simulink model "BLDC_SC_fr"  (R2021a)
settings: Solver=VariableStepAuto  StartTime=0.0  StopTime=3.5  MaxStep=1e-5  RelTol=1e-3
undefined symbols (not defined in the file or in its folder): B, DiscIntNeverNeededParam, J, Ke, Ls, p, pm, Rs, sigbuilder_block
libraries: spsVoltageMeasurementLib x3, simulink x1, spsDCVoltageSourceLib x1, spsUniversalBridgeLib x1, spsPermanentMagnetSynchronousMachineLib x1, spspowerguiLib x1
settings Model: SimulationMode=accelerator  Creator=musta  LastModifiedBy=AHMED
settings DebuggingCC: UnderSpecifiedDimensionMsg=warning

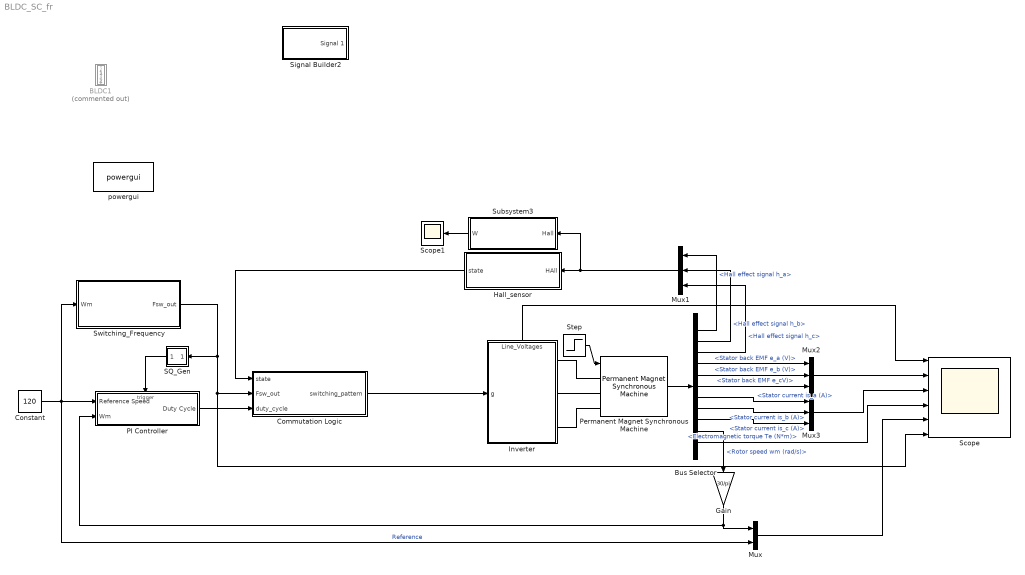
== system BLDC_SC_fr ==
  BLDC1 : Subsystem  Commented=on
  Bus Selector : BusSelector  OutputSignals=Hall effect signal h_a,Hall effect signal h_b,Hall effect signal h_c,Stator back EMF e_a (V),Stator back EMF e_b (V),Stator back EMF e_cV),Stator current is_a (A),Stator current is_b (A),Stator current is_c (A),Rotor speed wm (rad/s),Electromagnetic torque Te (N*m)
  Commutation Logic : Subsystem
  Constant : Constant  Value=120
  Gain : Gain  Gain=30/pi
  Hall_sensor : Subsystem
  Inverter : Subsystem
      settings: PortSchema="{\"entries\":[{\"content\":{\"sides\":[{\"content\":{\"connectorIds\":[\"In1\"]},\"type\":\"ConnectorPlacement.EquallySpacedRectSide\",\"uuid\":\"a4a631f5-5ca6-4816-ae34-76d65d1ebca4\"},{\"content\":{\"connectorIds\":[\"RConn1\",\"RConn2\",\"RConn3\"],\"side\":\"RIGHT\"},\"type\":\"ConnectorPlacement.EquallySpacedRectSide\",\"uuid\":\"fc2fa901-aafd-4005-bc6f-aa03a105cdb5\"},{\"content\":{\"connectorIds\":[\"Out1\"],\"side\":\"TOP\"},\"type\":\"ConnectorPlacement.EquallySpacedRectSide\",\"uuid\":\"9f3df2e4-0b81-43f4-a3b4-b6a902391765\"}]},\"type\":\"ConnectorPlacement.EquallySpacedConnector\",\"uuid\":\"eba0ffe2-2f10-412b-af1b-cd169af8270e\"}],\"packageUris\":[\"http://schema.mathworks.com/mf0/Connector/R2020b\"],\"version\":\"1.0\"}"
  Mux : Mux  Inputs=2
  Mux1 : Mux  Inputs=3
  Mux2 : Mux  Inputs=3
  Mux3 : Mux  Inputs=3
  PI Controller : Subsystem
  Permanent Magnet Synchronous Machine : spsPermanentMagnetSynchronousMachineLib/Permanent Magnet Synchronous Machine  NbPhases=3  FluxDistribution=Trapezoidal  RotorType=Round  MechanicalLoad=Torque Tm  PresetModel=No  ShowDetailedParameters=on  MeasurementBus=off  Resistance=0.1  Inductance=0.0018  dqInductances=[8.5e-3,8.5e-3]  La=0.0018  MachineConstant=Torque Constant (N.m / A_peak)  Flux=0.0034375  VoltageCst=17.2788  TorqueCst=0.165  Flat=120  Mechanical=[0.000621417 0.000303448 24]  PolePairs=4  InitialConditions=[0,0, 0,0]  InitialConditions5ph=[0 0 0 0 0 0]  RefAngle=Aligned with phase A axis (original Park)  IterativeDiscreteModel=Trapezoidal non iterative  TsBlock=-1  TsPowergui=0
  SQ_Gen : Subsystem
  Scope : Scope  NumInputPorts=6
  Scope1 : Scope
  Signal Builder2 : Subsystem  Tag=STV Subsys  LoadFcn=sigbuilder_block('load');  StartFcn=sigbuilder_block('start');  StopFcn=sigbuilder_block('stop');  ClipboardFcn=sigbuilder_block('clipboard');  mask(Sigbuilder block){tuvar=[0:10]}
      mask help: Simulink:masks:SigbuilderBlock_MD
      mask init:
      | if ~strcmp(get_param(bdroot(gcbh),'SimulationStatus'),'stopped') tuvar = sigbuilder_block('maskInit'); end
      settings: CopyFcn=sigbuilder_block('copy');  DeleteFcn=sigbuilder_block('delete');  ModelCloseFcn=sigbuilder_block('modelClose');  PreSaveFcn=sigbuilder_block('preSave');  PauseFcn=sigbuilder_block('pause');  ContinueFcn=sigbuilder_block('continue');  NameChangeFcn=sigbuilder_block('namechange');  OpenFcn=sigbuilder_block('open',[5.4 30 1141.2 522.6 ]);  CloseFcn=sigbuilder_block('close');
      mask Display: plot(0, 0, 100, 100,[2, 2, 32, 32, 2], [68, 8, 8, 68, 68],[32, 2], [38, 38], [32, 19, 2],[53, 60, 44], [32, 17, 17, 2],[16, 16, 31, 31]);txt = getActiveGroup(gcbh);text(2, 100, txt,'verticalAlignment', 'top');
  Step : Step  Time=1.25  After=0  SampleTime=0
  Subsystem3 : Subsystem
  Switching_Frequency : Subsystem
  powergui : spspowerguiLib/powergui  Priority=1  SimulationMode=Continuous  SampleTime=1e-6  frequency=60  Iterations=50  frequencyindice=0  Pbase=100e6  ErrMax=1e-4  UnitsV=kV  UnitsW=MW  buscounter=0  FunctionMessages=off  echomessages=off  EnableUseOfTLC=off  CurrentSourceSwitches=off  DisableSnubberDevices=off  DisableRonSwitches=off  DisableVfSwitches=off  DisplayEquations=off  AutomaticDiscreteSolvers=off  SolverType=Tustin/Backward Euler (TBE)  Interpol=off  ExternalGateDelay=off  methode=off  Ts=100  x0status=blocks  SPID=on  SwTol=0  HookPort=off  NonlinearTolerance=1e-4  nMaxIteration=100  ContinueOnMaxIteration=off  RestoreLinks=warning  ResistiveCurrentMeasurement=off  Frange=[0:2:500]  Ylog=off  Xlog=on  ShowGrid=off  save=off  variable=ZData  structure=0  ZoomFFT=off  StartTime=0.0  cycles=1  DisplayStyle=1  fundamental=60  FreqAxis=off  MaxFrequency=1000  frequencyindicesteady=1  RmsSteady=1  display=off
  wires:
  Hall_sensor/1(state) -> Commutation Logic/1("state ")
  PI Controller/1(Duty Cycle) -> Commutation Logic/3(duty_cycle)
  Switching_Frequency/1(Fsw_out) -> Scope/6, Commutation Logic/2(Fsw_out), SQ_Gen/1(Input)
  SQ_Gen/1(Cs) -> PI Controller/Trigger
  Permanent Magnet Synchronous Machine/1 -> Bus Selector/1
  Bus Selector/1 -> Mux1/1  "<Hall effect signal h_a>"
  Bus Selector/2 -> Mux1/2  "<Hall effect signal h_b>"
  Bus Selector/3 -> Mux1/3  "<Hall effect signal h_c>"
  Bus Selector/4 -> Mux2/1  "<Stator back EMF e_a (V)>"
  Bus Selector/5 -> Mux2/2  "<Stator back EMF e_b (V)>"
  Bus Selector/6 -> Mux2/3  "<Stator back EMF e_cV)>"
  Mux2/1 -> Scope/2
  Bus Selector/7 -> Mux3/1  "<Stator current is_a (A)>"
  Bus Selector/8 -> Mux3/2  "<Stator current is_b (A)>"
  Bus Selector/9 -> Mux3/3  "<Stator current is_c (A)>"
  Mux3/1 -> Scope/3
  Bus Selector/10 -> Gain/1  "<Rotor speed wm (rad/s)>"
  Bus Selector/11 -> Scope/4  "<Electromagnetic torque Te (N*m)>"
  Mux/1 -> Scope/5
  Step/1 -> Permanent Magnet Synchronous Machine/1
  Inverter/1(Line_Voltages) -> Scope/1
  Commutation Logic/1("  switching_pattern") -> Inverter/1(g)
  Constant/1 -> Switching_Frequency/1(Wm), Mux/2, PI Controller/1(Reference Speed)  "Reference"
  Mux1/1 -> Subsystem3/1(Hall), Hall_sensor/1(HAll)
  Gain/1 -> PI Controller/2(Wm), Mux/1
  Subsystem3/1(W) -> Scope1/1
  connections:
  Inverter/RConn1 -- Permanent Magnet Synchronous Machine/LConn1
  Inverter/RConn2 -- Permanent Magnet Synchronous Machine/LConn2
  Inverter/RConn3 -- Permanent Magnet Synchronous Machine/LConn3

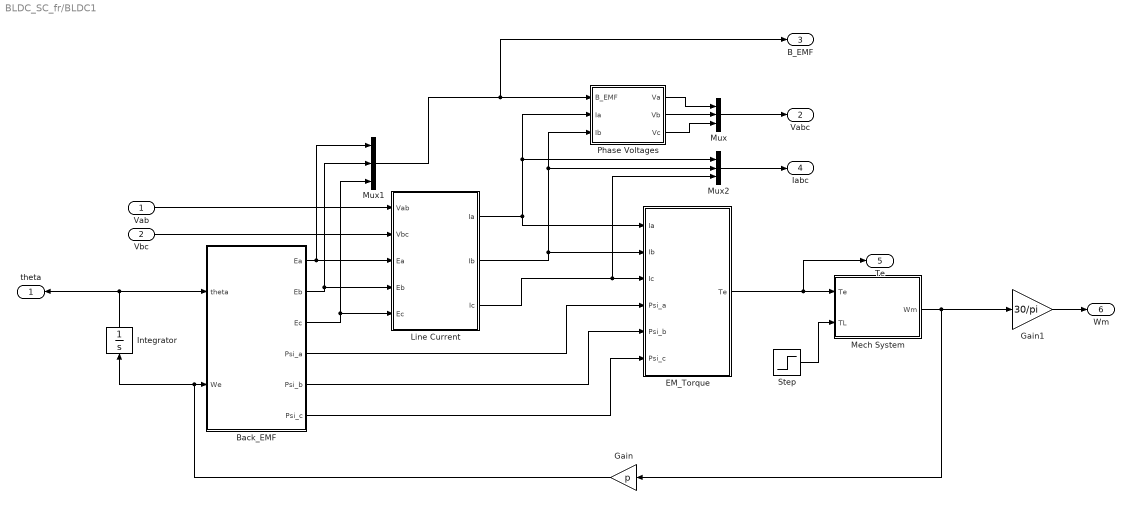
== system BLDC_SC_fr/BLDC1 ==
  Vab : Inport
  Vbc : Inport  Port=2
  Back_EMF : Subsystem
  EM_Torque : Subsystem
  Gain : Gain  Gain=p
  Gain1 : Gain  Gain=30/pi
  Integrator : Integrator
  Line Current : Subsystem
  Mech System : Subsystem
  Mux : Mux  Inputs=3
  Mux1 : Mux  Inputs=3
  Mux2 : Mux  Inputs=3
  Phase Voltages : Subsystem
  Step : Step  Time=2.5  Before=0.5  After=1.5  SampleTime=0
  theta : Outport
  Vabc : Outport  Port=2
  B_EMF : Outport  Port=3
  Iabc : Outport  Port=4
  Te : Outport  Port=5
  Wm : Outport  Port=6
  wires:
  Integrator/1 -> Back_EMF/1(theta), theta/1
  Mux2/1 -> Iabc/1
  Mux/1 -> Vabc/1
  Phase Voltages/3(Vc) -> Mux/3
  Phase Voltages/2(Vb) -> Mux/2
  Phase Voltages/1(Va) -> Mux/1
  Line Current/1(Ia) -> Phase Voltages/2(Ia), Mux2/1, EM_Torque/1(Ia)
  Gain1/1 -> Wm/1
  Vbc/1 -> Line Current/2(Vbc)
  Step/1 -> Mech System/2(TL)
  Vab/1 -> Line Current/1(Vab)
  Mux1/1 -> Phase Voltages/1(B_EMF), B_EMF/1
  Back_EMF/4(Psi_a) -> EM_Torque/4(Psi_a)
  Line Current/2(Ib) -> EM_Torque/2(Ib), Phase Voltages/3(Ib), Mux2/2
  Back_EMF/5(Psi_b) -> EM_Torque/5(Psi_b)
  Gain/1 -> Back_EMF/2(We), Integrator/1
  Back_EMF/6(Psi_c) -> EM_Torque/6(Psi_c)
  EM_Torque/1(Te) -> Mech System/1(Te), Te/1
  Back_EMF/2(Eb) -> Line Current/4(Eb), Mux1/2
  Back_EMF/3(Ec) -> Mux1/3, Line Current/5(Ec)
  Line Current/3(Ic) -> EM_Torque/3(Ic), Mux2/3
  Back_EMF/1(Ea) -> Line Current/3(Ea), Mux1/1
  Mech System/1(Wm) -> Gain/1, Gain1/1

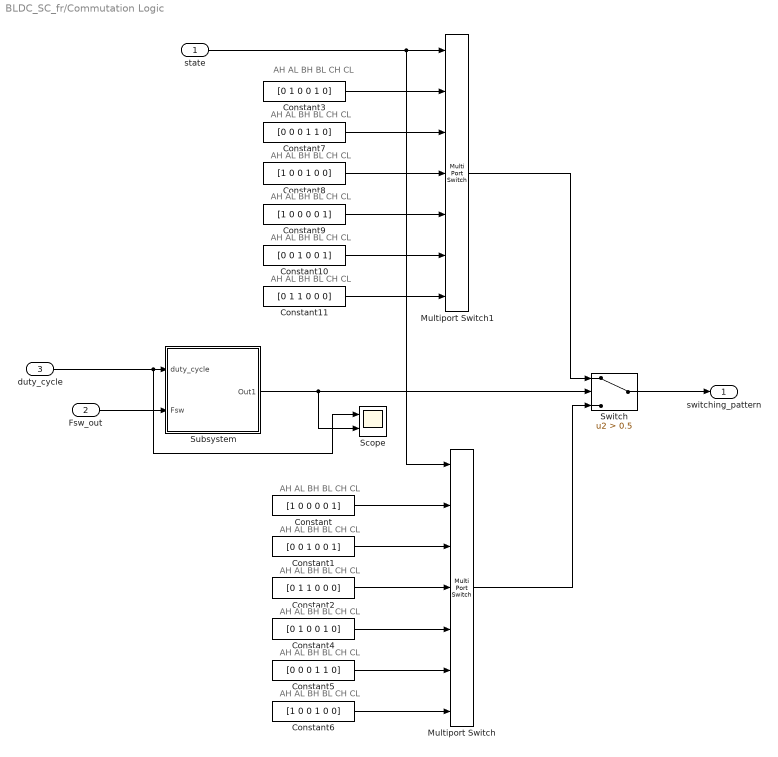
== system BLDC_SC_fr/Commutation Logic ==
  note: AH AL BH BL CH CL
  note: AH AL BH BL CH CL
  note: AH AL BH BL CH CL
  note: AH AL BH BL CH CL
  note: AH AL BH BL CH CL
  note: AH AL BH BL CH CL
  note: AH AL BH BL CH CL
  note: AH AL BH BL CH CL
  note: AH AL BH BL CH CL
  note: AH AL BH BL CH CL
  note: AH AL BH BL CH CL
  note: AH AL BH BL CH CL
  "state " : Inport
  Fsw_out : Inport  Port=2
  duty_cycle : Inport  Port=3
  Constant : Constant  Value=[1 0 0 0 0 1]
  Constant1 : Constant  Value=[0 0 1 0 0 1]
  Constant10 : Constant  Value=[0 0 1 0 0 1]
  Constant11 : Constant  Value=[0 1 1 0 0 0]
  Constant2 : Constant  Value=[0 1 1 0 0 0]
  Constant3 : Constant  Value=[0 1 0 0 1 0]
  Constant4 : Constant  Value=[0 1 0 0 1 0]
  Constant5 : Constant  Value=[0 0 0 1 1 0]
  Constant6 : Constant  Value=[1 0 0 1 0 0]
  Constant7 : Constant  Value=[0 0 0 1 1 0]
  Constant8 : Constant  Value=[1 0 0 1 0 0]
  Constant9 : Constant  Value=[1 0 0 0 0 1]
  Multiport Switch : MultiPortSwitch  Inputs=6
  Multiport Switch1 : MultiPortSwitch  Inputs=6
  Scope : Scope  NumInputPorts=2
  Subsystem : Subsystem
  Switch : Switch  Criteria=u2 > Threshold  Threshold=0.5
  "  switching_pattern" : Outport  VectorParamsAs1DForOutWhenUnconnected=off
  wires:
  Constant1/1 -> Multiport Switch/3
  Constant11/1 -> Multiport Switch1/7
  Constant2/1 -> Multiport Switch/4
  Constant10/1 -> Multiport Switch1/6
  Constant/1 -> Multiport Switch/2
  Switch/1 -> "  switching_pattern"/1
  Constant9/1 -> Multiport Switch1/5
  Constant7/1 -> Multiport Switch1/3
  Constant6/1 -> Multiport Switch/7
  Constant3/1 -> Multiport Switch1/2
  Constant8/1 -> Multiport Switch1/4
  Constant4/1 -> Multiport Switch/5
  Constant5/1 -> Multiport Switch/6
  "state "/1 -> Multiport Switch/1, Multiport Switch1/1
  Multiport Switch1/1 -> Switch/1
  Multiport Switch/1 -> Switch/3
  duty_cycle/1 -> Scope/1, Subsystem/1(duty_cycle)
  Fsw_out/1 -> Subsystem/2(Fsw)
  Subsystem/1(Out1) -> Scope/2, Switch/2

== system BLDC_SC_fr/Hall_sensor ==
  HAll : Inport
  Demux : Demux  Outputs=3
  MATLAB Function : MATLAB Function  TreatAsAtomicUnit=on
  state : Outport
  wires:
  HAll/1 -> Demux/1
  Demux/1 -> MATLAB Function/1(H1)
  Demux/2 -> MATLAB Function/2(H2)
  Demux/3 -> MATLAB Function/3(H3)
  MATLAB Function/1(State) -> state/1

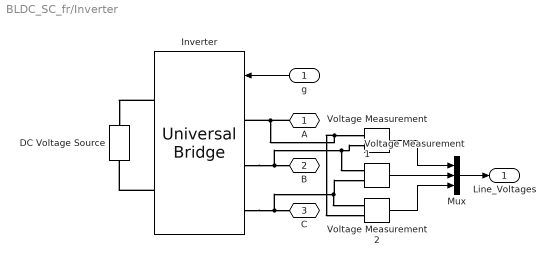
== system BLDC_SC_fr/Inverter ==
  g : Inport
  DC Voltage Source : spsDCVoltageSourceLib/DC Voltage Source  Amplitude=48  Measurements=None
  Inverter : spsUniversalBridgeLib/Universal Bridge  Arms=3  SnubberResistance=1e5  SnubberCapacitance=inf  Device=IGBT / Diodes  Ron=1e-3  Lon=0  ForwardVoltages="[  0  0  ]"  ForwardVoltage=0  GTOparameters=[ 10e-6 , 20e-6 ]  IGBTparameters=[ 1e-6 , 2e-6 ]  Measurements=None  Measurements_2=None  converterType=Rectifier
  Mux : Mux  Inputs=3
  Voltage Measurement : spsVoltageMeasurementLib/Voltage Measurement  PhasorSimulation=off  OutputType=Complex  PSBequivalent=0
  Voltage Measurement1 : spsVoltageMeasurementLib/Voltage Measurement  PhasorSimulation=off  OutputType=Complex  PSBequivalent=0
  Voltage Measurement2 : spsVoltageMeasurementLib/Voltage Measurement  PhasorSimulation=off  OutputType=Complex  PSBequivalent=0
  A : PMIOPort  Side=Right
  B : PMIOPort  Port=2  Side=Right
  C : PMIOPort  Port=3  Side=Right
  Line_Voltages : Outport
  wires:
  g/1 -> Inverter/1
  Voltage Measurement/1 -> Mux/1
  Voltage Measurement1/1 -> Mux/2
  Voltage Measurement2/1 -> Mux/3
  Mux/1 -> Line_Voltages/1
  connections:
  Inverter/RConn1 -- DC Voltage Source/RConn1
  Inverter/RConn2 -- DC Voltage Source/LConn1
  A/RConn1 -- Voltage Measurement/LConn1 -- Voltage Measurement2/LConn2 -- Inverter/LConn1
  Inverter/LConn2 -- Voltage Measurement1/LConn1 -- Voltage Measurement/LConn2 -- B/RConn1
  Inverter/LConn3 -- Voltage Measurement2/LConn1 -- Voltage Measurement1/LConn2 -- C/RConn1

== system BLDC_SC_fr/PI Controller ==
  Reference Speed : Inport
  Wm : Inport  Port=2
  Trigger : TriggerPort  VariantControl=(inherit)  PortDimensions=1
  PI_system3 : Subsystem
  Sum : Sum  Inputs=|+-
  Duty Cycle : Outport
  wires:
  Sum/1 -> PI_system3/1(Error)
  PI_system3/1(T_ref) -> Duty Cycle/1
  Wm/1 -> Sum/2
  Reference Speed/1 -> Sum/1

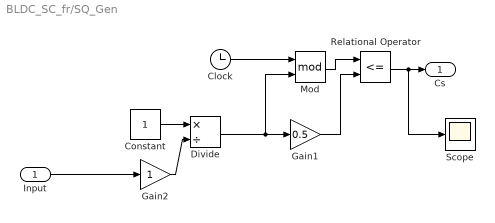
== system BLDC_SC_fr/SQ_Gen ==
  Input : Inport
  Clock : Clock
  Constant : Constant
  Divide : Product  Inputs=*/
  Gain1 : Gain  Gain=0.5
  Gain2 : Gain
  Mod : Math  Operator=mod  SaturateOnIntegerOverflow=on
  Relational Operator : RelationalOperator  Operator=<=  OutDataTypeStr=boolean  RndMeth=Simplest
  Scope : Scope
  Cs : Outport
  wires:
  Input/1 -> Gain2/1
  Clock/1 -> Mod/1
  Mod/1 -> Relational Operator/1
  Gain2/1 -> Divide/2
  Divide/1 -> Gain1/1, Mod/2
  Constant/1 -> Divide/1
  Gain1/1 -> Relational Operator/2
  Relational Operator/1 -> Scope/1, Cs/1

== system BLDC_SC_fr/Signal Builder2 ==
  Demux : Demux  Tag=STV Demux  Outputs=1
      settings: DisplayOption=none
  FromWs : FromWorkspace  Tag=STV FromWs  VariableName=tuvar  SampleTime=-1
      SigBuilderData=|
      | common.afterFinalStr = 'Extrapolate'
      | common.sampleTime = '-1'
      | dataSet.timeRange = [0 3.5]
      | dataSet.name = 'Group 1'
      | sbobj.Groups.Name = 'Group 1'
      | sbobj.Groups.Signals.Name = 'Signal 1'
      | sbobj.Groups.Signals.XData = [0 0.25 0.5 1 1.5 1.75 2 2.5 2.75 3 3.5]
      | sbobj.Groups.Signals.YData = [0.25 0.5 0.5 1.5 1.5 2 1.5 1.5 0.5 0.25 0.25]
      | sbobj.Groups.TimeRange = [0 3.5]
  Signal 1 : Outport  Tag=STV Outport
  wires:
  FromWs/1 -> Demux/1
  Demux/1 -> Signal 1/1

== system BLDC_SC_fr/Subsystem3 ==
  Hall : Inport
  Add : Sum  Inputs=+++
  Demux : Demux  Outputs=3
  Gain2 : Gain  Gain=1/3
  Scope1 : Scope  NumInputPorts=4
  Subsystem : Subsystem
  Subsystem1 : Subsystem
  Subsystem2 : Subsystem
  W : Outport
  wires:
  Subsystem2/1(Out1) -> Add/1
  Demux/3 -> Subsystem/1(U)
  Subsystem/1(Out1) -> Add/3
  Demux/2 -> Subsystem1/1(U)
  Add/1 -> Gain2/1
  Subsystem1/1(Out1) -> Add/2
  Demux/1 -> Subsystem2/1(U)
  Hall/1 -> Demux/1
  Gain2/1 -> W/1

== system BLDC_SC_fr/Switching_Frequency ==
  Wm : Inport
  Gain : Gain  Gain=10
  Gain1 : Gain  Gain=1/500
  Gain2 : Gain  Gain=500
  N2F : Gain  Gain=48/120
  Round : Rounding  Operator=round
  Saturation : Saturate  UpperLimit=10000  LowerLimit=4000
  Wm2N : Gain  Gain=60/(2*pi)
  Fsw_out : Outport
  wires:
  Wm2N/1 -> N2F/1
  Wm/1 -> Wm2N/1
  N2F/1 -> Gain/1
  Saturation/1 -> Gain1/1
  Gain1/1 -> Round/1
  Gain2/1 -> Fsw_out/1
  Round/1 -> Gain2/1
  Gain/1 -> Saturation/1

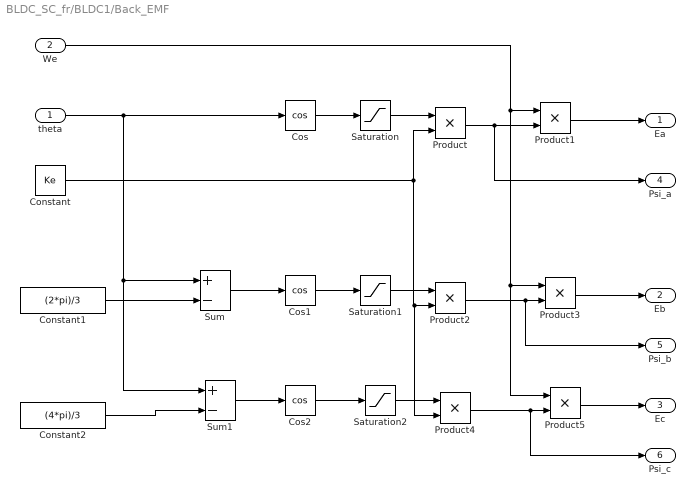
== system BLDC_SC_fr/BLDC1/Back_EMF ==
  theta : Inport
  We : Inport  Port=2
  Constant : Constant  Value=Ke
  Constant1 : Constant  Value=(2*pi)/3
  Constant2 : Constant  Value=(4*pi)/3
  Cos : Trigonometry  Operator=cos
  Cos1 : Trigonometry  Operator=cos
  Cos2 : Trigonometry  Operator=cos
  Product{,1..5} (6 alike) : Product
  Saturation : Saturate
  Saturation1 : Saturate
  Saturation2 : Saturate
  Sum : Sum  Inputs=+-
  Sum1 : Sum  Inputs=+-
  Ea : Outport
  Eb : Outport  Port=2
  Ec : Outport  Port=3
  Psi_a : Outport  Port=4
  Psi_b : Outport  Port=5
  Psi_c : Outport  Port=6
  wires:
  Product5/1 -> Ec/1
  Constant2/1 -> Sum1/2
  Sum1/1 -> Cos2/1
  Cos2/1 -> Saturation2/1
  Saturation2/1 -> Product4/1
  Product4/1 -> Product5/2, Psi_c/1
  Product3/1 -> Eb/1
  Product2/1 -> Product3/2, Psi_b/1
  Saturation1/1 -> Product2/1
  Cos1/1 -> Saturation1/1
  Sum/1 -> Cos1/1
  Constant1/1 -> Sum/2
  Constant/1 -> Product/2, Product2/2, Product4/2
  Product1/1 -> Ea/1
  We/1 -> Product1/1, Product3/1, Product5/1
  Product/1 -> Product1/2, Psi_a/1
  Saturation/1 -> Product/1
  Cos/1 -> Saturation/1
  theta/1 -> Sum/1, Sum1/1, Cos/1

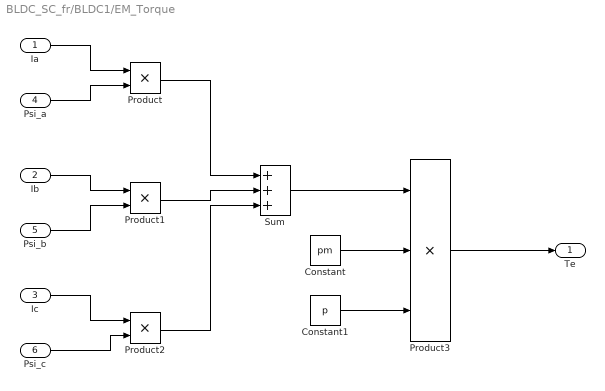
== system BLDC_SC_fr/BLDC1/EM_Torque ==
  Ia : Inport
  Ib : Inport  Port=2
  Ic : Inport  Port=3
  Psi_a : Inport  Port=4
  Psi_b : Inport  Port=5
  Psi_c : Inport  Port=6
  Constant : Constant  Value=pm
  Constant1 : Constant  Value=p
  Product : Product
  Product1 : Product
  Product2 : Product
  Product3 : Product  Inputs=3
  Sum : Sum  Inputs=+++
  Te : Outport
  wires:
  Product3/1 -> Te/1
  Constant1/1 -> Product3/3
  Constant/1 -> Product3/2
  Sum/1 -> Product3/1
  Product2/1 -> Sum/3
  Product1/1 -> Sum/2
  Product/1 -> Sum/1
  Psi_c/1 -> Product2/2
  Ic/1 -> Product2/1
  Psi_b/1 -> Product1/2
  Ib/1 -> Product1/1
  Psi_a/1 -> Product/2
  Ia/1 -> Product/1

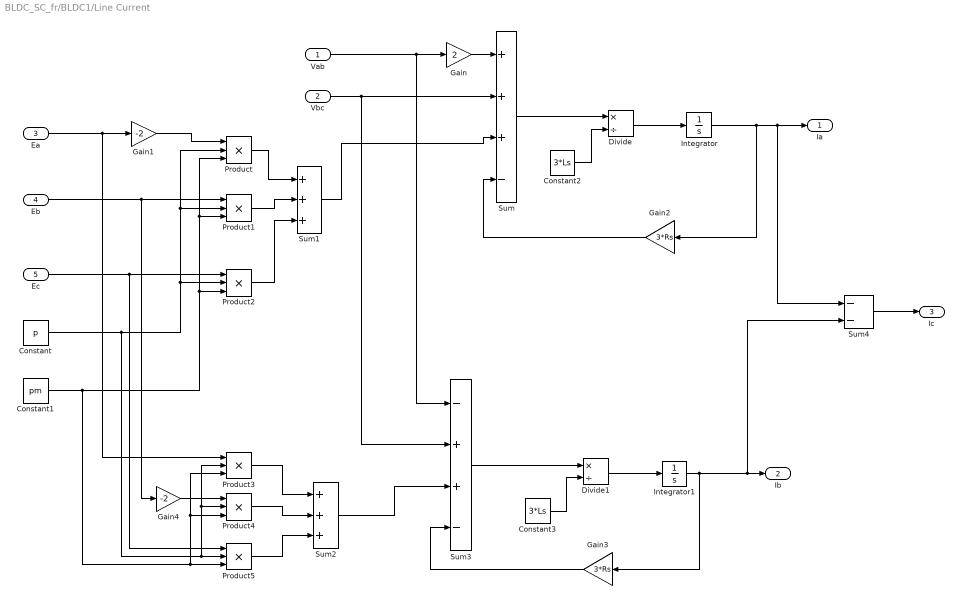
== system BLDC_SC_fr/BLDC1/Line Current ==
  Vab : Inport
  Vbc : Inport  Port=2
  Ea : Inport  Port=3
  Eb : Inport  Port=4
  Ec : Inport  Port=5
  Constant : Constant  Value=p
  Constant1 : Constant  Value=pm
  Constant2 : Constant  Value=3*Ls
  Constant3 : Constant  Value=3*Ls
  Divide : Product  Inputs=*/
  Divide1 : Product  Inputs=*/
  Gain : Gain  Gain=2
  Gain1 : Gain  Gain=-2
  Gain2 : Gain  Gain=3*Rs
  Gain3 : Gain  Gain=3*Rs
  Gain4 : Gain  Gain=-2
  Integrator : Integrator
  Integrator1 : Integrator
  Product{,1..5} (6 alike) : Product  Inputs=3
  Sum : Sum  Inputs=+++-
  Sum1 : Sum  Inputs=+++
  Sum2 : Sum  Inputs=+++
  Sum3 : Sum  Inputs=-++-
  Sum4 : Sum  Inputs=--
  Ia : Outport
  Ib : Outport  Port=2
  Ic : Outport  Port=3
  wires:
  Gain4/1 -> Product4/1
  Sum4/1 -> Ic/1
  Gain3/1 -> Sum3/4
  Integrator1/1 -> Ib/1, Sum4/2, Gain3/1
  Sum3/1 -> Divide1/1
  Constant3/1 -> Divide1/2
  Divide1/1 -> Integrator1/1
  Sum2/1 -> Sum3/3
  Product5/1 -> Sum2/3
  Product4/1 -> Sum2/2
  Product3/1 -> Sum2/1
  Gain2/1 -> Sum/4
  Integrator/1 -> Ia/1, Sum4/1, Gain2/1
  Divide/1 -> Integrator/1
  Constant2/1 -> Divide/2
  Sum/1 -> Divide/1
  Sum1/1 -> Sum/3
  Product2/1 -> Sum1/3
  Product1/1 -> Sum1/2
  Product/1 -> Sum1/1
  Constant1/1 -> Product2/3, Product/3, Product1/3, Product5/3, Product4/3, Product3/3
  Constant/1 -> Product2/2, Product/2, Product1/2, Product5/2, Product4/2, Product3/2
  Ec/1 -> Product2/1, Product5/1
  Eb/1 -> Product1/1, Gain4/1
  Gain1/1 -> Product/1
  Ea/1 -> Gain1/1, Product3/1
  Vbc/1 -> Sum/2, Sum3/2
  Gain/1 -> Sum/1
  Vab/1 -> Gain/1, Sum3/1

== system BLDC_SC_fr/BLDC1/Mech System ==
  Te : Inport
  TL : Inport  Port=2
  Constant : Constant  Value=J
  Divide : Product  Inputs=*/
  Gain : Gain  Gain=B
  Integrator : Integrator
  Sum : Sum  Inputs=+--
  Wm : Outport
  wires:
  Gain/1 -> Sum/3
  Integrator/1 -> Wm/1, Gain/1
  Divide/1 -> Integrator/1
  Constant/1 -> Divide/2
  Sum/1 -> Divide/1
  TL/1 -> Sum/2
  Te/1 -> Sum/1

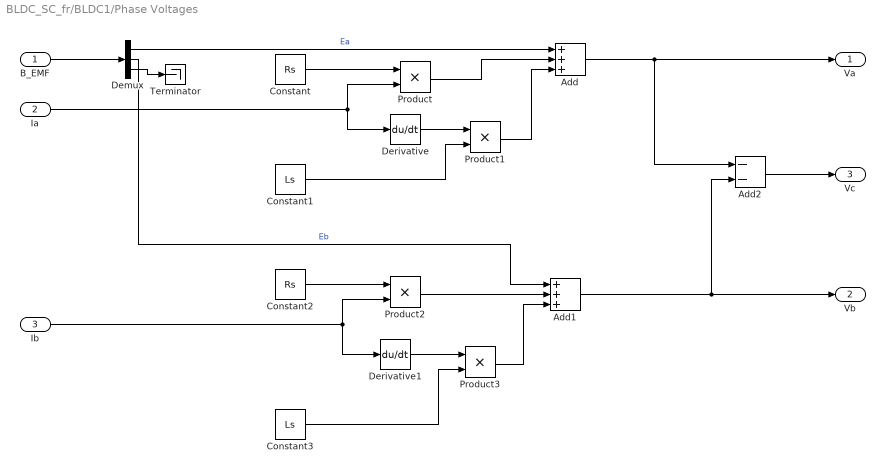
== system BLDC_SC_fr/BLDC1/Phase Voltages ==
  B_EMF : Inport
  Ia : Inport  Port=2
  Ib : Inport  Port=3
  Add : Sum  Inputs=+++
  Add1 : Sum  Inputs=+++
  Add2 : Sum  Inputs=--
  Constant : Constant  Value=Rs
  Constant1 : Constant  Value=Ls
  Constant2 : Constant  Value=Rs
  Constant3 : Constant  Value=Ls
  Demux : Demux  Outputs=3
  Derivative : Derivative
  Derivative1 : Derivative
  Product{,1..3} (4 alike) : Product
  Terminator : Terminator
  Va : Outport
  Vb : Outport  Port=2
  Vc : Outport  Port=3
  wires:
  Add2/1 -> Vc/1
  Constant3/1 -> Product3/2
  Constant2/1 -> Product2/1
  Constant1/1 -> Product1/2
  Constant/1 -> Product/1
  Demux/3 -> Terminator/1
  Add1/1 -> Vb/1, Add2/2
  Demux/2 -> Add1/1  "Eb"
  Product2/1 -> Add1/2
  Derivative1/1 -> Product3/1
  Product3/1 -> Add1/3
  Ib/1 -> Product2/2, Derivative1/1
  Demux/1 -> Add/1  "Ea"
  B_EMF/1 -> Demux/1
  Ia/1 -> Product/2, Derivative/1
  Product1/1 -> Add/3
  Add/1 -> Va/1, Add2/1
  Derivative/1 -> Product1/1
  Product/1 -> Add/2

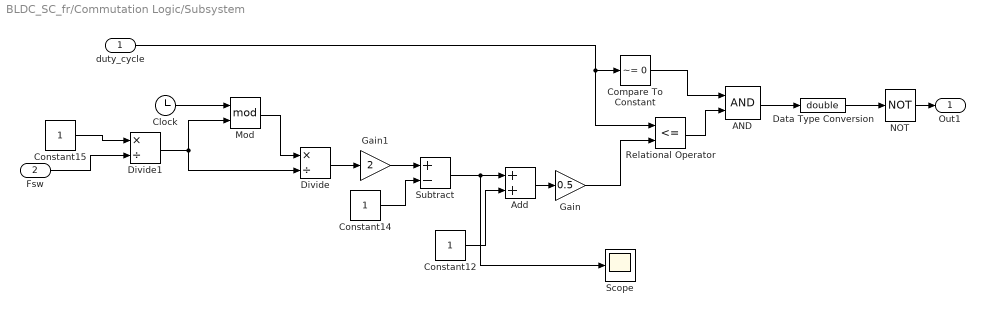
== system BLDC_SC_fr/Commutation Logic/Subsystem ==
  duty_cycle : Inport
  Fsw : Inport  Port=2
  AND : Logic  AllPortsSameDT=off  OutDataTypeStr=boolean
  Add : Sum
  Clock : Clock
  Compare To Constant : simulink/Logic and Bit Operations/Compare To Constant  relop=~=  const=0  OutDataTypeStr=boolean
  Constant12 : Constant
  Constant14 : Constant
  Constant15 : Constant
  Data Type Conversion : DataTypeConversion  OutDataTypeStr=double
  Divide : Product  Inputs=*/
  Divide1 : Product  Inputs=*/
  Gain : Gain  Gain=0.5
  Gain1 : Gain  Gain=2
  Mod : Math  Operator=mod  SaturateOnIntegerOverflow=on
  NOT : Logic  Operator=NOT  IconShape=distinctive  AllPortsSameDT=off  OutDataTypeStr=boolean
  Relational Operator : RelationalOperator  Operator=<=  OutDataTypeStr=boolean  RndMeth=Simplest
  Scope : Scope
  Subtract : Sum  Inputs=+-
  Out1 : Outport
  wires:
  Constant12/1 -> Add/2
  Add/1 -> Gain/1
  Relational Operator/1 -> AND/2
  Constant14/1 -> Subtract/2
  NOT/1 -> Out1/1
  duty_cycle/1 -> Relational Operator/1, Compare To Constant/1
  Subtract/1 -> Scope/1, Add/1
  Compare To Constant/1 -> AND/1
  Gain/1 -> Relational Operator/2
  AND/1 -> Data Type Conversion/1
  Divide1/1 -> Divide/2, Mod/2
  Gain1/1 -> Subtract/1
  Clock/1 -> Mod/1
  Mod/1 -> Divide/1
  Divide/1 -> Gain1/1
  Constant15/1 -> Divide1/1
  Fsw/1 -> Divide1/2
  Data Type Conversion/1 -> NOT/1

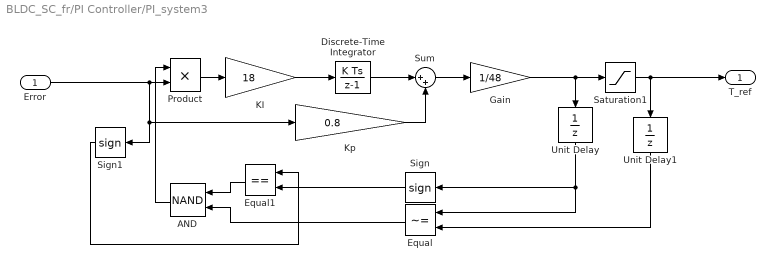
== system BLDC_SC_fr/PI Controller/PI_system3 ==
  Error : Inport
  AND : Logic  Operator=NAND  AllPortsSameDT=off  OutDataTypeStr=boolean
  Discrete-Time Integrator : DiscreteIntegrator  SampleTime=-1  ICPrevOutput=DiscIntNeverNeededParam  ICPrevScaledInput=DiscIntNeverNeededParam
  Equal : RelationalOperator  Operator=~=  OutDataTypeStr=boolean  RndMeth=Simplest
  Equal1 : RelationalOperator  Operator===  OutDataTypeStr=boolean  RndMeth=Simplest
  Gain : Gain  Gain=1/48
  KI : Gain  Gain=18
  Kp : Gain  Gain=0.8
  Product : Product
  Saturation1 : Saturate  UpperLimit=1  LowerLimit=0
  Sign : Signum
  Sign1 : Signum
  Sum : Sum  Inputs=|++
  Unit Delay : UnitDelay  SampleTime=-1  HasFrameUpgradeWarning=on
  Unit Delay1 : UnitDelay  SampleTime=-1  HasFrameUpgradeWarning=on
  T_ref : Outport
  wires:
  Error/1 -> Kp/1, Sign1/1, Product/2
  AND/1 -> Product/1
  Unit Delay1/1 -> Equal/2
  Product/1 -> KI/1
  Unit Delay/1 -> Equal/1, Sign/1
  Equal/1 -> AND/2
  Equal1/1 -> AND/1
  Sign1/1 -> Equal1/1
  Sign/1 -> Equal1/2
  Saturation1/1 -> Unit Delay1/1, T_ref/1
  Sum/1 -> Gain/1
  KI/1 -> Discrete-Time Integrator/1
  Kp/1 -> Sum/2
  Discrete-Time Integrator/1 -> Sum/1
  Gain/1 -> Saturation1/1, Unit Delay/1

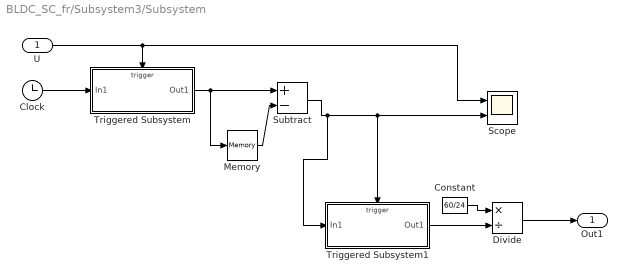
== system BLDC_SC_fr/Subsystem3/Subsystem ==
  U : Inport
  Clock : Clock
  Constant : Constant  Value=60/24
  Divide : Product  Inputs=*/
  Memory : Memory  InheritSampleTime=on
  Scope : Scope  NumInputPorts=2
  Subtract : Sum  Inputs=+-
  Triggered Subsystem : Subsystem  TreatAsAtomicUnit=on
  Triggered Subsystem1 : Subsystem  TreatAsAtomicUnit=on
  Out1 : Outport
  wires:
  Clock/1 -> Triggered Subsystem/1(In1)
  Subtract/1 -> Triggered Subsystem1/1(In1), Triggered Subsystem1/Trigger, Scope/2
  Triggered Subsystem/1(Out1) -> Subtract/1, Memory/1
  Memory/1 -> Subtract/2
  U/1 -> Triggered Subsystem/Trigger, Scope/1
  Triggered Subsystem1/1(Out1) -> Divide/2
  Constant/1 -> Divide/1
  Divide/1 -> Out1/1

== system BLDC_SC_fr/Subsystem3/Subsystem1 ==
  U : Inport
  Clock : Clock
  Constant : Constant  Value=60/24
  Divide : Product  Inputs=*/
  Memory : Memory  InheritSampleTime=on
  Scope : Scope  NumInputPorts=2
  Subtract : Sum  Inputs=+-
  Triggered Subsystem : Subsystem  TreatAsAtomicUnit=on
  Triggered Subsystem1 : Subsystem  TreatAsAtomicUnit=on
  Out1 : Outport
  wires:
  Divide/1 -> Out1/1
  Constant/1 -> Divide/1
  Triggered Subsystem1/1(Out1) -> Divide/2
  U/1 -> Scope/1, Triggered Subsystem/Trigger
  Memory/1 -> Subtract/2
  Triggered Subsystem/1(Out1) -> Memory/1, Subtract/1
  Subtract/1 -> Scope/2, Triggered Subsystem1/Trigger, Triggered Subsystem1/1(In1)
  Clock/1 -> Triggered Subsystem/1(In1)

== system BLDC_SC_fr/Subsystem3/Subsystem2 ==
  U : Inport
  Clock : Clock
  Constant : Constant  Value=60/24
  Divide : Product  Inputs=*/
  Memory : Memory  InheritSampleTime=on
  Scope : Scope  NumInputPorts=2
  Subtract : Sum  Inputs=+-
  Triggered Subsystem : Subsystem  TreatAsAtomicUnit=on
  Triggered Subsystem1 : Subsystem  TreatAsAtomicUnit=on
  Out1 : Outport
  wires:
  Clock/1 -> Triggered Subsystem/1(In1)
  Subtract/1 -> Triggered Subsystem1/1(In1), Triggered Subsystem1/Trigger, Scope/2
  Triggered Subsystem/1(Out1) -> Subtract/1, Memory/1
  Memory/1 -> Subtract/2
  U/1 -> Triggered Subsystem/Trigger, Scope/1
  Triggered Subsystem1/1(Out1) -> Divide/2
  Constant/1 -> Divide/1
  Divide/1 -> Out1/1

== system BLDC_SC_fr/Subsystem3/Subsystem/Triggered Subsystem ==
  In1 : Inport
  Trigger : TriggerPort  VariantControl=(inherit)
  Out1 : Outport
  wires:
  In1/1 -> Out1/1

== system BLDC_SC_fr/Subsystem3/Subsystem/Triggered Subsystem1 ==
  In1 : Inport
  Trigger : TriggerPort  VariantControl=(inherit)
  Out1 : Outport
  wires:
  In1/1 -> Out1/1

== system BLDC_SC_fr/Subsystem3/Subsystem1/Triggered Subsystem ==
  In1 : Inport
  Trigger : TriggerPort  VariantControl=(inherit)
  Out1 : Outport
  wires:
  In1/1 -> Out1/1

== system BLDC_SC_fr/Subsystem3/Subsystem1/Triggered Subsystem1 ==
  In1 : Inport
  Trigger : TriggerPort  VariantControl=(inherit)
  Out1 : Outport
  wires:
  In1/1 -> Out1/1

== system BLDC_SC_fr/Subsystem3/Subsystem2/Triggered Subsystem ==
  In1 : Inport
  Trigger : TriggerPort  VariantControl=(inherit)
  Out1 : Outport
  wires:
  In1/1 -> Out1/1

== system BLDC_SC_fr/Subsystem3/Subsystem2/Triggered Subsystem1 ==
  In1 : Inport
  Trigger : TriggerPort  VariantControl=(inherit)
  Out1 : Outport
  wires:
  In1/1 -> Out1/1

== matlab function BLDC_SC_fr/Hall_sensor/MATLAB Function ==
  data: H1 input; State output; H2 input; H3 input
function State = fcn(H1,H2,H3)

State = 0 ;
if H1 == 0 && H2 == 0 && H3 == 1 
    State = 1;
elseif H1 == 1 && H2 == 0 && H3 == 1 
    State = 2;
elseif H1 == 1 && H2 == 0 && H3 == 0 
    State = 3;
elseif H1 == 1 && H2 == 1 && H3 == 0
    State = 4;
elseif H1 == 0 && H2 == 1 && H3 == 0
    State = 5;
elseif H1 == 0 && H2 == 1 && H3 == 1
    State = 6;
end
end
